simulink model "fullWaveBridgeRectifier_threePhase"  (R2024b)
settings: Solver=VariableStepAuto  StartTime=0.0  StopTime=0.1  RelTol=1e-3
libraries: fl_lib x3, ee_lib x2, nesl_utility x1
settings Model: Creator=farha  LastModifiedBy=farha

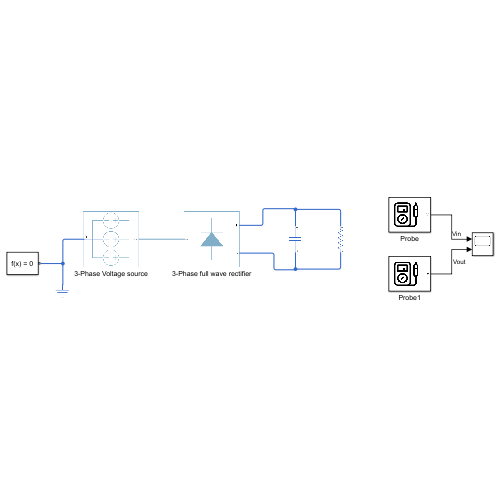
[thumbnail: Simulink's stored preview of the top-level diagram]
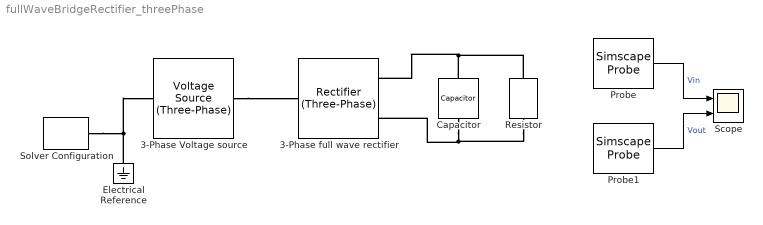
== system fullWaveBridgeRectifier_threePhase ==
  3-Phase Voltage source : ee_lib/Sources/Voltage Source (Three-Phase)  vline_rms=208 V  shift=120 deg  freq=60 Hz  impedance_option=0  SShortCircuit=1e6 A*V  XR=15  R=0.01 Ohm  L=3.97e-4 H  harmonic_option=0  harmonic_orders=[5, 7, 11, 13]  harmonic_ratios=[.1, .1, .1, .1]  G_parasitic=0 1/Ohm  I_specify=off  I_priority=None  I=[0, 0, 0] A  I_nominal_specify=off  I_nominal_value=1  I_nominal_unit=A
  3-Phase full wave rectifier : ee_lib/Semiconductors & Converters/Converters/Rectifier (Three-Phase)  port_option=ee.enum.threePhasePort.composite  Vf=0.8 V  Ron=0.001 Ohm  Goff=1e-5 1/Ohm  model_dynamics=ee.enum.converters.diode.nodynamics  C=50 nF  iRM=-235 A  iF=300 A  idot=-50 A/us  trr_param=ee.enum.converters.diodetrr.trr_factor  trr_factor=3  trr=15 us  Qrr=1500 s*uA
      settings: InternalSimscapePortConfiguration="{\"Bottom\":[],\"Left\":[{\"id\":\"N\",\"label\":\"~\",\"type\":\"foundation.electrical.three_phase\"}],\"Right\":[{\"id\":\"p\",\"label\":\"+\",\"type\":\"foundation.electrical.electrical\"},{\"id\":\"n\",\"label\":\"-\",\"type\":\"foundation.electrical.electrical\"}],\"Top\":[]}"
  Capacitor : fl_lib/Electrical/Electrical Elements/Capacitor  c=10 mF  r=1e-6 Ohm  g=0 1/Ohm  i_specify=off  i_priority=None  i=0 A  i_nominal_specify=off  i_nominal_value=1  i_nominal_unit=A  v_specify=off  v_priority=None  v=0 V  v_nominal_specify=off  v_nominal_value=1  v_nominal_unit=V  vc_specify=off  vc_priority=High  vc=0 V  vc_nominal_specify=off  vc_nominal_value=1  vc_nominal_unit=V
  Electrical Reference : fl_lib/Electrical/Electrical Elements/Electrical Reference
  Probe : SimscapeProbe  BoundBlock=1  Variables="{\"V\":{\"Unit\":\"V\",\"PortLabel\":\"V\",\"Probing\":\"ON\"}}"
  Probe1 : SimscapeProbe  BoundBlock=9  Variables="{\"v\":{\"Unit\":\"V\",\"PortLabel\":\"v\",\"Probing\":\"ON\"}}"
  Resistor : fl_lib/Electrical/Electrical Elements/Resistor  R=400 Ohm  i_specify=off  i_priority=None  i=0 A  i_nominal_specify=off  i_nominal_value=1  i_nominal_unit=A  v_specify=off  v_priority=None  v=0 V  v_nominal_specify=off  v_nominal_value=1  v_nominal_unit=V
  Scope : Scope  NumInputPorts=2
  Solver Configuration : nesl_utility/Solver Configuration  PhysicalDomain=network_engine_domain  SubClassName=solver  LeftPortType=input  RightPortType=generic  Tones=[]  Harmonics=[]  SimulateNoise=off  Profile=off  UseLocalSampling=off  EnableSwitchedLinearOptims=on  FrequencyDomain=off  UseCCode=off  RelTol=0.001  AbsTol=0.001  MinStep=1e-09  ToWorkspace=off  RevertToSquareIcSolve=off  NumHomotopyIterations=100  PhasorMode=off  PhasorModeNumHarmonics=1  ConsistencySolver=NEWTON_XTOL_AFTER_FTOL  IndexReductionMethod=DerivativeReplacement  DoDC=off  ResidualTolerance=1e-09  ConsistencyTolSource=GLOBAL  ConsistencyAbsTol=0.001  ConsistencyRelTol=0.001  ConsistencyTolFactor=0.001  UseLocalSolver=off  LocalSolverChoice=NE_BACKWARD_EULER_ADVANCER  ResolveIndetEquations=on  FunctionEvalNumThread=1  LocalSolverSampleTime=0.001  DoFixedCost=off  MaxNonlinIter=3  MaxModeIter=2  ComputeImpulses=off  ImpulseIterations=2  LinearAlgebra=auto  LinearAlgebraNumThread=0  EquationFormulation=NE_TIME_EF  DelaysMemoryBudget=1024  AutomaticFiltering=on  FilteringTimeConstant=0.001  PartitionStorageMethod=AS_NEEDED  PartitionMemoryBudget=1024  PartitionMethod=ROBUST  MultibodyUseLocalSolver=off  MultibodyLocalSolverChoice=ODE1  MultibodyLocalSolverSampleTime=0.001
  wires:
  Probe/1 -> Scope/1  "Vin"
  Probe1/1 -> Scope/2  "Vout"
  connections:
  Electrical Reference/LConn1 -- Solver Configuration/RConn1 -- 3-Phase Voltage source/LConn1
  3-Phase Voltage source/RConn1 -- 3-Phase full wave rectifier/LConn1
  Capacitor/LConn1 -- Resistor/LConn1 -- 3-Phase full wave rectifier/RConn1
  Capacitor/RConn1 -- Resistor/RConn1 -- 3-Phase full wave rectifier/RConn2
